simulink model "DPWMA_17_Level_Rectifier_Dual_PI"  (R2021b)
settings: Solver=VariableStepAuto  StartTime=0.0  StopTime=0.5  RelTol=1e-3
libraries: spsSeriesRLCBranchLib x51, spsVoltageMeasurementLib x27, spsDiodeLib x24, spsIGBTDiodeLib x24, simulink x24, spsUniversalBridgeLib x24, slpidlib x3, spsACVoltageSourceLib x3, spsCurrentMeasurementLib x2, spsMeanLib x2, spsRMSLib x2, spsTHDLib x1
(part 2 of 3)

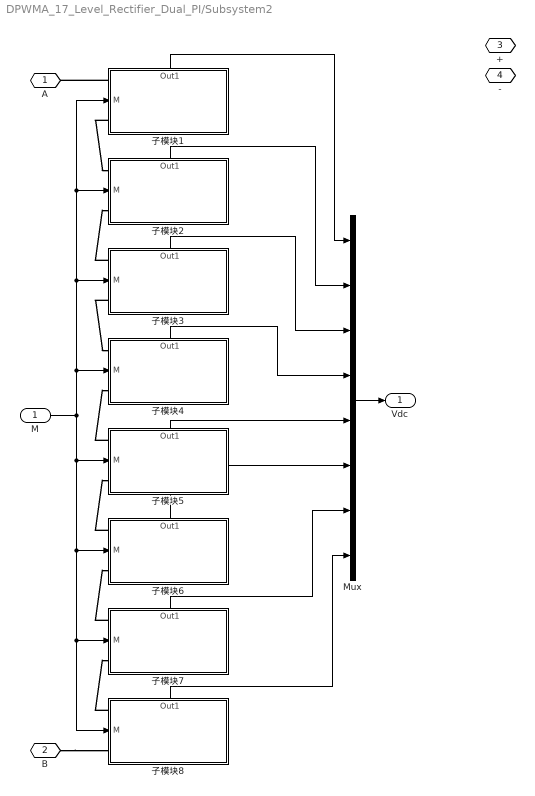
== system DPWMA_17_Level_Rectifier_Dual_PI/Subsystem2 ==
  M : Inport
  Mux : Mux  Inputs=8
  子模块1 : Subsystem
      settings: PortSchema="{\"entries\":[{\"content\":{\"sides\":[{\"content\":{\"connectorIds\":[\"LConn1\",\"LConn2\"]},\"type\":\"ConnectorPlacement.EquallySpacedRectSide\",\"uuid\":\"47187a24-6853-42ac-9ad9-0df0e1360fae\"},{\"content\":{\"connectorIds\":[\"RConn1\",\"In1\",\"RConn2\"],\"side\":\"RIGHT\"},\"type\":\"ConnectorPlacement.EquallySpacedRectSide\",\"uuid\":\"b3504369-b235-4116-9b9b-167bd6b76527\"},{\"content\":{\"connectorIds\":[\"Out1\"],\"side\":\"TOP\"},\"type\":\"ConnectorPlacement.EquallySpacedRectSide\",\"uuid\":\"5cb205b4-da18-4f20-b3d4-22846a9c2236\"},{\"content\":{\"connectorIds\":[],\"side\":\"BOTTOM\"},\"type\":\"ConnectorPlacement.EquallySpacedRectSide\",\"uuid\":\"4e548a82-6bdf-470e-8572-00c7c8855d01\"}]},\"type\":\"ConnectorPlacement.EquallySpacedConnector\",\"uuid\":\"b00ba750-ea4b-4b64-a122-5cbc9e899126\"}],\"packageUris\":[\"http://schema.mathworks.com/mf0/Connector/R2020b\"],\"version\":\"1.0\"}"
  子模块2 : Subsystem
      settings: PortSchema="{\"entries\":[{\"content\":{\"sides\":[{\"content\":{\"connectorIds\":[\"LConn1\",\"LConn2\"]},\"type\":\"ConnectorPlacement.EquallySpacedRectSide\",\"uuid\":\"47187a24-6853-42ac-9ad9-0df0e1360fae\"},{\"content\":{\"connectorIds\":[\"RConn1\",\"In1\",\"RConn2\"],\"side\":\"RIGHT\"},\"type\":\"ConnectorPlacement.EquallySpacedRectSide\",\"uuid\":\"b3504369-b235-4116-9b9b-167bd6b76527\"},{\"content\":{\"connectorIds\":[\"Out1\"],\"side\":\"TOP\"},\"type\":\"ConnectorPlacement.EquallySpacedRectSide\",\"uuid\":\"5cb205b4-da18-4f20-b3d4-22846a9c2236\"},{\"content\":{\"connectorIds\":[],\"side\":\"BOTTOM\"},\"type\":\"ConnectorPlacement.EquallySpacedRectSide\",\"uuid\":\"4e548a82-6bdf-470e-8572-00c7c8855d01\"}]},\"type\":\"ConnectorPlacement.EquallySpacedConnector\",\"uuid\":\"b00ba750-ea4b-4b64-a122-5cbc9e899126\"}],\"packageUris\":[\"http://schema.mathworks.com/mf0/Connector/R2020b\"],\"version\":\"1.0\"}"
  子模块3 : Subsystem
      settings: PortSchema="{\"entries\":[{\"content\":{\"sides\":[{\"content\":{\"connectorIds\":[\"LConn1\",\"LConn2\"]},\"type\":\"ConnectorPlacement.EquallySpacedRectSide\",\"uuid\":\"47187a24-6853-42ac-9ad9-0df0e1360fae\"},{\"content\":{\"connectorIds\":[\"RConn1\",\"In1\",\"RConn2\"],\"side\":\"RIGHT\"},\"type\":\"ConnectorPlacement.EquallySpacedRectSide\",\"uuid\":\"b3504369-b235-4116-9b9b-167bd6b76527\"},{\"content\":{\"connectorIds\":[\"Out1\"],\"side\":\"TOP\"},\"type\":\"ConnectorPlacement.EquallySpacedRectSide\",\"uuid\":\"5cb205b4-da18-4f20-b3d4-22846a9c2236\"},{\"content\":{\"connectorIds\":[],\"side\":\"BOTTOM\"},\"type\":\"ConnectorPlacement.EquallySpacedRectSide\",\"uuid\":\"4e548a82-6bdf-470e-8572-00c7c8855d01\"}]},\"type\":\"ConnectorPlacement.EquallySpacedConnector\",\"uuid\":\"b00ba750-ea4b-4b64-a122-5cbc9e899126\"}],\"packageUris\":[\"http://schema.mathworks.com/mf0/Connector/R2020b\"],\"version\":\"1.0\"}"
  子模块4 : Subsystem
      settings: PortSchema="{\"entries\":[{\"content\":{\"sides\":[{\"content\":{\"connectorIds\":[\"LConn1\",\"LConn2\"]},\"type\":\"ConnectorPlacement.EquallySpacedRectSide\",\"uuid\":\"47187a24-6853-42ac-9ad9-0df0e1360fae\"},{\"content\":{\"connectorIds\":[\"RConn1\",\"In1\",\"RConn2\"],\"side\":\"RIGHT\"},\"type\":\"ConnectorPlacement.EquallySpacedRectSide\",\"uuid\":\"b3504369-b235-4116-9b9b-167bd6b76527\"},{\"content\":{\"connectorIds\":[\"Out1\"],\"side\":\"TOP\"},\"type\":\"ConnectorPlacement.EquallySpacedRectSide\",\"uuid\":\"5cb205b4-da18-4f20-b3d4-22846a9c2236\"},{\"content\":{\"connectorIds\":[],\"side\":\"BOTTOM\"},\"type\":\"ConnectorPlacement.EquallySpacedRectSide\",\"uuid\":\"4e548a82-6bdf-470e-8572-00c7c8855d01\"}]},\"type\":\"ConnectorPlacement.EquallySpacedConnector\",\"uuid\":\"b00ba750-ea4b-4b64-a122-5cbc9e899126\"}],\"packageUris\":[\"http://schema.mathworks.com/mf0/Connector/R2020b\"],\"version\":\"1.0\"}"
  子模块5 : Subsystem
      settings: PortSchema="{\"entries\":[{\"content\":{\"sides\":[{\"content\":{\"connectorIds\":[\"LConn1\",\"LConn2\"]},\"type\":\"ConnectorPlacement.EquallySpacedRectSide\",\"uuid\":\"47187a24-6853-42ac-9ad9-0df0e1360fae\"},{\"content\":{\"connectorIds\":[\"RConn1\",\"In1\",\"RConn2\"],\"side\":\"RIGHT\"},\"type\":\"ConnectorPlacement.EquallySpacedRectSide\",\"uuid\":\"b3504369-b235-4116-9b9b-167bd6b76527\"},{\"content\":{\"connectorIds\":[\"Out1\"],\"side\":\"TOP\"},\"type\":\"ConnectorPlacement.EquallySpacedRectSide\",\"uuid\":\"5cb205b4-da18-4f20-b3d4-22846a9c2236\"},{\"content\":{\"connectorIds\":[],\"side\":\"BOTTOM\"},\"type\":\"ConnectorPlacement.EquallySpacedRectSide\",\"uuid\":\"4e548a82-6bdf-470e-8572-00c7c8855d01\"}]},\"type\":\"ConnectorPlacement.EquallySpacedConnector\",\"uuid\":\"b00ba750-ea4b-4b64-a122-5cbc9e899126\"}],\"packageUris\":[\"http://schema.mathworks.com/mf0/Connector/R2020b\"],\"version\":\"1.0\"}"
  子模块6 : Subsystem
      settings: PortSchema="{\"entries\":[{\"content\":{\"sides\":[{\"content\":{\"connectorIds\":[\"LConn1\",\"LConn2\"]},\"type\":\"ConnectorPlacement.EquallySpacedRectSide\",\"uuid\":\"47187a24-6853-42ac-9ad9-0df0e1360fae\"},{\"content\":{\"connectorIds\":[\"RConn1\",\"In1\",\"RConn2\"],\"side\":\"RIGHT\"},\"type\":\"ConnectorPlacement.EquallySpacedRectSide\",\"uuid\":\"b3504369-b235-4116-9b9b-167bd6b76527\"},{\"content\":{\"connectorIds\":[\"Out1\"],\"side\":\"TOP\"},\"type\":\"ConnectorPlacement.EquallySpacedRectSide\",\"uuid\":\"5cb205b4-da18-4f20-b3d4-22846a9c2236\"},{\"content\":{\"connectorIds\":[],\"side\":\"BOTTOM\"},\"type\":\"ConnectorPlacement.EquallySpacedRectSide\",\"uuid\":\"4e548a82-6bdf-470e-8572-00c7c8855d01\"}]},\"type\":\"ConnectorPlacement.EquallySpacedConnector\",\"uuid\":\"b00ba750-ea4b-4b64-a122-5cbc9e899126\"}],\"packageUris\":[\"http://schema.mathworks.com/mf0/Connector/R2020b\"],\"version\":\"1.0\"}"
  子模块7 : Subsystem
      settings: PortSchema="{\"entries\":[{\"content\":{\"sides\":[{\"content\":{\"connectorIds\":[\"LConn1\",\"LConn2\"]},\"type\":\"ConnectorPlacement.EquallySpacedRectSide\",\"uuid\":\"47187a24-6853-42ac-9ad9-0df0e1360fae\"},{\"content\":{\"connectorIds\":[\"RConn1\",\"In1\",\"RConn2\"],\"side\":\"RIGHT\"},\"type\":\"ConnectorPlacement.EquallySpacedRectSide\",\"uuid\":\"b3504369-b235-4116-9b9b-167bd6b76527\"},{\"content\":{\"connectorIds\":[\"Out1\"],\"side\":\"TOP\"},\"type\":\"ConnectorPlacement.EquallySpacedRectSide\",\"uuid\":\"5cb205b4-da18-4f20-b3d4-22846a9c2236\"},{\"content\":{\"connectorIds\":[],\"side\":\"BOTTOM\"},\"type\":\"ConnectorPlacement.EquallySpacedRectSide\",\"uuid\":\"4e548a82-6bdf-470e-8572-00c7c8855d01\"}]},\"type\":\"ConnectorPlacement.EquallySpacedConnector\",\"uuid\":\"b00ba750-ea4b-4b64-a122-5cbc9e899126\"}],\"packageUris\":[\"http://schema.mathworks.com/mf0/Connector/R2020b\"],\"version\":\"1.0\"}"
  子模块8 : Subsystem
      settings: PortSchema="{\"entries\":[{\"content\":{\"sides\":[{\"content\":{\"connectorIds\":[\"LConn1\",\"LConn2\"]},\"type\":\"ConnectorPlacement.EquallySpacedRectSide\",\"uuid\":\"47187a24-6853-42ac-9ad9-0df0e1360fae\"},{\"content\":{\"connectorIds\":[\"RConn1\",\"In1\",\"RConn2\"],\"side\":\"RIGHT\"},\"type\":\"ConnectorPlacement.EquallySpacedRectSide\",\"uuid\":\"b3504369-b235-4116-9b9b-167bd6b76527\"},{\"content\":{\"connectorIds\":[\"Out1\"],\"side\":\"TOP\"},\"type\":\"ConnectorPlacement.EquallySpacedRectSide\",\"uuid\":\"5cb205b4-da18-4f20-b3d4-22846a9c2236\"},{\"content\":{\"connectorIds\":[],\"side\":\"BOTTOM\"},\"type\":\"ConnectorPlacement.EquallySpacedRectSide\",\"uuid\":\"4e548a82-6bdf-470e-8572-00c7c8855d01\"}]},\"type\":\"ConnectorPlacement.EquallySpacedConnector\",\"uuid\":\"b00ba750-ea4b-4b64-a122-5cbc9e899126\"}],\"packageUris\":[\"http://schema.mathworks.com/mf0/Connector/R2020b\"],\"version\":\"1.0\"}"
  A : PMIOPort  Side=Left
  B : PMIOPort  Port=2  Side=Left
  + : PMIOPort  Port=3  Side=Right
  - : PMIOPort  Port=4  Side=Right
  Vdc : Outport
  wires:
  子模块3/1(Out1) -> Mux/3
  子模块1/1(Out1) -> Mux/1
  子模块2/1(Out1) -> Mux/2
  子模块4/1(Out1) -> Mux/4
  Mux/1 -> Vdc/1
  M/1 -> 子模块8/1(M), 子模块7/1(M), 子模块6/1(M), 子模块5/1(M), 子模块1/1(M), 子模块2/1(M), 子模块3/1(M), 子模块4/1(M)
  子模块8/1(Out1) -> Mux/8
  子模块6/1(Out1) -> Mux/6
  子模块7/1(Out1) -> Mux/7
  子模块5/1(Out1) -> Mux/5
  connections:
  子模块1/RConn2 -- 子模块2/RConn1
  子模块1/RConn1 -- A/RConn1
  子模块3/RConn1 -- 子模块2/RConn2
  子模块3/RConn2 -- 子模块4/RConn1
  B/RConn1 -- 子模块8/RConn2
  子模块8/RConn1 -- 子模块7/RConn2
  子模块7/RConn1 -- 子模块6/RConn2
  子模块6/RConn1 -- 子模块5/RConn2
  子模块5/RConn1 -- 子模块4/RConn2

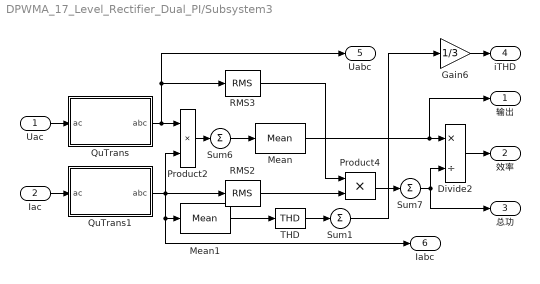
== system DPWMA_17_Level_Rectifier_Dual_PI/Subsystem3 ==
  Uac : Inport
  Iac : Inport  Port=2
  Divide2 : Product  Inputs=*/
  Gain6 : Gain  Gain=1/3
  Mean : spsMeanLib/Mean  Freq=100  Vinit=0  Ts=0
  Mean1 : spsMeanLib/Mean  Freq=20000  Vinit=0  Ts=0
  Product2 : Product
  Product4 : Product
  QuTrans : Subsystem
      settings: PortSchema="{\"entries\":[{\"content\":{\"sides\":[{\"content\":{\"connectorIds\":[]},\"type\":\"ConnectorPlacement.EquallySpacedRectSide\",\"uuid\":\"58c40194-9a95-4e39-952e-f878bde7484e\"},{\"content\":{\"connectorIds\":[],\"side\":\"RIGHT\"},\"type\":\"ConnectorPlacement.EquallySpacedRectSide\",\"uuid\":\"f51692e8-3ff2-4d72-808d-3667196a4526\"},{\"content\":{\"connectorIds\":[\"In1\"],\"side\":\"TOP\"},\"type\":\"ConnectorPlacement.EquallySpacedRectSide\",\"uuid\":\"0aab136b-5da5-45c4-8998-999ebe8b7f2f\"},{\"content\":{\"connectorIds\":[\"Out1\"],\"side\":\"BOTTOM\"},\"type\":\"ConnectorPlacement.EquallySpacedRectSide\",\"uuid\":\"185ce796-68e2-4136-8080-97dc86d2ba54\"}]},\"type\":\"ConnectorPlacement.EquallySpacedConnector\",\"uuid\":\"3ef81af7-d426-47fb-88e3-e33e58eebb83\"}],\"packageUris\":[\"http://schema.mathworks.com/mf0/Connector/R2020b\"],\"version\":\"1.0\"}"
  QuTrans1 : Subsystem
      settings: PortSchema="{\"entries\":[{\"content\":{\"sides\":[{\"content\":{\"connectorIds\":[]},\"type\":\"ConnectorPlacement.EquallySpacedRectSide\",\"uuid\":\"58c40194-9a95-4e39-952e-f878bde7484e\"},{\"content\":{\"connectorIds\":[],\"side\":\"RIGHT\"},\"type\":\"ConnectorPlacement.EquallySpacedRectSide\",\"uuid\":\"f51692e8-3ff2-4d72-808d-3667196a4526\"},{\"content\":{\"connectorIds\":[\"In1\"],\"side\":\"TOP\"},\"type\":\"ConnectorPlacement.EquallySpacedRectSide\",\"uuid\":\"0aab136b-5da5-45c4-8998-999ebe8b7f2f\"},{\"content\":{\"connectorIds\":[\"Out1\"],\"side\":\"BOTTOM\"},\"type\":\"ConnectorPlacement.EquallySpacedRectSide\",\"uuid\":\"185ce796-68e2-4136-8080-97dc86d2ba54\"}]},\"type\":\"ConnectorPlacement.EquallySpacedConnector\",\"uuid\":\"3ef81af7-d426-47fb-88e3-e33e58eebb83\"}],\"packageUris\":[\"http://schema.mathworks.com/mf0/Connector/R2020b\"],\"version\":\"1.0\"}"
  RMS2 : spsRMSLib/RMS  TrueRMS=on  Freq=50  RMSInit=0  Ts=0
  RMS3 : spsRMSLib/RMS  TrueRMS=on  Freq=50  RMSInit=0  Ts=0
  Sum1 : Sum  Inputs=+
  Sum6 : Sum  Inputs=+
  Sum7 : Sum  Inputs=+
  THD : spsTHDLib/THD  Freq=50  Ts=0
      settings: SourceProductBaseCode=PS
  输出 : Outport
  效率 : Outport  Port=2
  总功 : Outport  Port=3
  iTHD : Outport  Port=4
  Uabc : Outport  Port=5
  Iabc : Outport  Port=6
  wires:
  RMS3/1 -> Product4/1
  Product4/1 -> Sum7/1
  Sum6/1 -> Mean/1
  Product2/1 -> Sum6/1
  Divide2/1 -> 效率/1
  RMS2/1 -> Product4/2
  Sum1/1 -> Gain6/1
  Gain6/1 -> iTHD/1
  Sum7/1 -> 总功/1, Divide2/2
  Mean/1 -> 输出/1, Divide2/1
  THD/1 -> Sum1/1
  Mean1/1 -> THD/1
  Uac/1 -> QuTrans/1(ac)
  Iac/1 -> QuTrans1/1(ac)
  QuTrans1/1(abc) -> Product2/2, Iabc/1, Mean1/1, RMS2/1
  QuTrans/1(abc) -> Uabc/1, RMS3/1, Product2/1

== system DPWMA_17_Level_Rectifier_Dual_PI/三相电源 ==
  5.7KV2 : spsACVoltageSourceLib/AC Voltage Source  Amplitude=5770*1.414  Phase=120  Frequency=50  SampleTime=0  Measurements=None  BusType=swing  Pref=10e3  Qref=0  Qmin=-inf  Qmax=+inf
  5.7kV : spsACVoltageSourceLib/AC Voltage Source  Amplitude=5770*1.414  Phase=0  Frequency=50  SampleTime=0  Measurements=None  BusType=swing  Pref=10e3  Qref=0  Qmin=-inf  Qmax=+inf
  5.7kV1 : spsACVoltageSourceLib/AC Voltage Source  Amplitude=5770*1.414  Phase=240  Frequency=50  SampleTime=0  Measurements=None  BusType=swing  Pref=10e3  Qref=0  Qmin=-inf  Qmax=+inf
  A : PMIOPort  Side=Right
  B : PMIOPort  Port=2  Side=Right
  C : PMIOPort  Port=3  Side=Right
  N : PMIOPort  Port=4  Side=Right
  connections:
  5.7kV/LConn1 -- N/RConn1 -- 5.7KV2/LConn1 -- 5.7kV1/LConn1
  A/RConn1 -- 5.7kV/RConn1
  B/RConn1 -- 5.7kV1/RConn1
  C/RConn1 -- 5.7KV2/RConn1

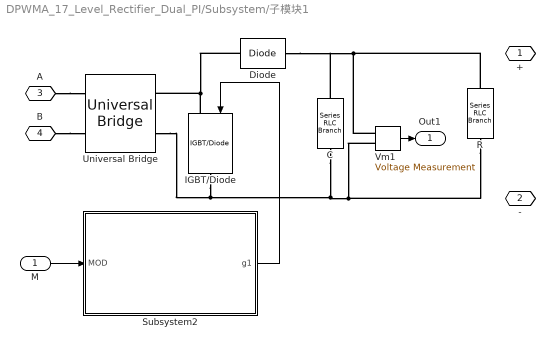
== system DPWMA_17_Level_Rectifier_Dual_PI/Subsystem/子模块1 ==
  M : Inport
  C : spsSeriesRLCBranchLib/Series RLC Branch  LConnTagsString=__new0  RConnTagsString=__new0  BranchType=C  Resistance=0  Inductance=0  SetiL0=off  InitialCurrent=0  Capacitance=4e-3  Setx0=on  InitialVoltage=1000  Measurements=None
  Diode : spsDiodeLib/Diode  Ron=0.001  Lon=0  Vf=2  IC=0  UseSnubber=0  Rs=1e6  Cs=2e-9  Measurements=off
  IGBT/Diode : spsIGBTDiodeLib/IGBT//Diode  Ron=1e-3  Rs=1e5  Cs=inf  Measurements=off
  R : spsSeriesRLCBranchLib/Series RLC Branch  LConnTagsString=__new0  RConnTagsString=__new0  BranchType=R  Resistance=15  Inductance=0  SetiL0=off  InitialCurrent=0  Capacitance=2e-3  Setx0=on  InitialVoltage=311  Measurements=None
  Subsystem2 : Subsystem
  Universal Bridge : spsUniversalBridgeLib/Universal Bridge  Arms=2  SnubberResistance=0.01  SnubberCapacitance=1e-8  Device=Diodes  Ron=1e-3  Lon=0  ForwardVoltages="[  0  0  ]"  ForwardVoltage=3  GTOparameters=[ 10e-6 , 20e-6 ]  IGBTparameters=[ 1e-6 , 2e-6 ]  Measurements=None  Measurements_2=None  converterType=Rectifier
  Vm1 : spsVoltageMeasurementLib/Voltage Measurement  PhasorSimulation=off  OutputType=Complex  PSBequivalent=0
  + : PMIOPort  Side=Left
  - : PMIOPort  Port=2  Side=Left
  A : PMIOPort  Port=3  Side=Right
  B : PMIOPort  Port=4  Side=Right
  Out1 : Outport
  wires:
  Vm1/1 -> Out1/1
  M/1 -> Subsystem2/1(MOD)
  Subsystem2/1(g1) -> IGBT/Diode/1
  connections:
  Universal Bridge/RConn2 -- Vm1/LConn2 -- R/RConn1 -- C/RConn1 -- IGBT/Diode/RConn1
  Vm1/LConn1 -- R/LConn1 -- C/LConn1 -- Diode/RConn1
  A/RConn1 -- Universal Bridge/LConn1
  B/RConn1 -- Universal Bridge/LConn2
  IGBT/Diode/LConn1 -- Universal Bridge/RConn1 -- Diode/LConn1

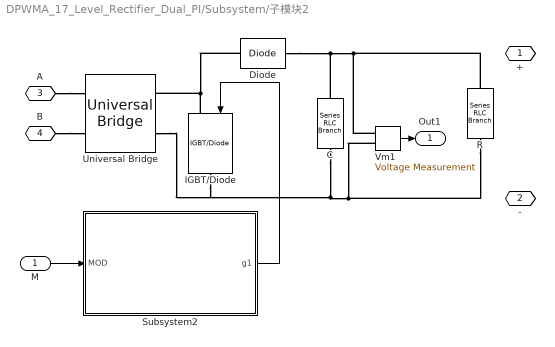
== system DPWMA_17_Level_Rectifier_Dual_PI/Subsystem/子模块2 ==
  M : Inport
  C : spsSeriesRLCBranchLib/Series RLC Branch  LConnTagsString=__new0  RConnTagsString=__new0  BranchType=C  Resistance=0  Inductance=0  SetiL0=off  InitialCurrent=0  Capacitance=4e-3  Setx0=on  InitialVoltage=1000  Measurements=None
  Diode : spsDiodeLib/Diode  Ron=0.001  Lon=0  Vf=2  IC=0  UseSnubber=0  Rs=1e6  Cs=2e-9  Measurements=off
  IGBT/Diode : spsIGBTDiodeLib/IGBT//Diode  Ron=1e-3  Rs=1e5  Cs=inf  Measurements=off
  R : spsSeriesRLCBranchLib/Series RLC Branch  LConnTagsString=__new0  RConnTagsString=__new0  BranchType=R  Resistance=15  Inductance=0  SetiL0=off  InitialCurrent=0  Capacitance=2e-3  Setx0=on  InitialVoltage=311  Measurements=None
  Subsystem2 : Subsystem
  Universal Bridge : spsUniversalBridgeLib/Universal Bridge  Arms=2  SnubberResistance=0.01  SnubberCapacitance=1e-8  Device=Diodes  Ron=1e-3  Lon=0  ForwardVoltages="[  0  0  ]"  ForwardVoltage=3  GTOparameters=[ 10e-6 , 20e-6 ]  IGBTparameters=[ 1e-6 , 2e-6 ]  Measurements=None  Measurements_2=None  converterType=Rectifier
  Vm1 : spsVoltageMeasurementLib/Voltage Measurement  PhasorSimulation=off  OutputType=Complex  PSBequivalent=0
  + : PMIOPort  Side=Left
  - : PMIOPort  Port=2  Side=Left
  A : PMIOPort  Port=3  Side=Right
  B : PMIOPort  Port=4  Side=Right
  Out1 : Outport
  wires:
  Vm1/1 -> Out1/1
  M/1 -> Subsystem2/1(MOD)
  Subsystem2/1(g1) -> IGBT/Diode/1
  connections:
  Vm1/LConn2 -- IGBT/Diode/RConn1 -- Universal Bridge/RConn2 -- C/RConn1 -- R/RConn1
  C/LConn1 -- Diode/RConn1 -- Vm1/LConn1 -- R/LConn1
  A/RConn1 -- Universal Bridge/LConn1
  B/RConn1 -- Universal Bridge/LConn2
  IGBT/Diode/LConn1 -- Diode/LConn1 -- Universal Bridge/RConn1

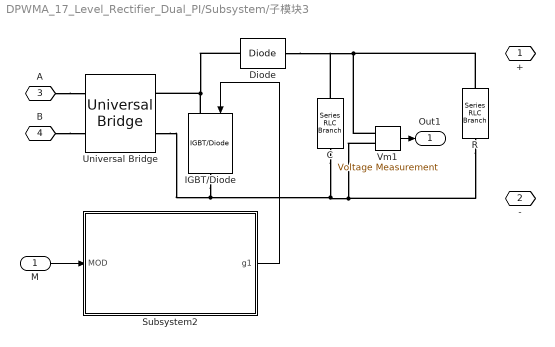
== system DPWMA_17_Level_Rectifier_Dual_PI/Subsystem/子模块3 ==
  M : Inport
  C : spsSeriesRLCBranchLib/Series RLC Branch  LConnTagsString=__new0  RConnTagsString=__new0  BranchType=C  Resistance=0  Inductance=0  SetiL0=off  InitialCurrent=0  Capacitance=4e-3  Setx0=on  InitialVoltage=1000  Measurements=None
  Diode : spsDiodeLib/Diode  Ron=0.001  Lon=0  Vf=2  IC=0  UseSnubber=0  Rs=1e6  Cs=2e-9  Measurements=off
  IGBT/Diode : spsIGBTDiodeLib/IGBT//Diode  Ron=1e-3  Rs=1e5  Cs=inf  Measurements=off
  R : spsSeriesRLCBranchLib/Series RLC Branch  LConnTagsString=__new0  RConnTagsString=__new0  BranchType=R  Resistance=15  Inductance=0  SetiL0=off  InitialCurrent=0  Capacitance=2e-3  Setx0=on  InitialVoltage=311  Measurements=None
  Subsystem2 : Subsystem
  Universal Bridge : spsUniversalBridgeLib/Universal Bridge  Arms=2  SnubberResistance=0.01  SnubberCapacitance=1e-8  Device=Diodes  Ron=1e-3  Lon=0  ForwardVoltages="[  0  0  ]"  ForwardVoltage=3  GTOparameters=[ 10e-6 , 20e-6 ]  IGBTparameters=[ 1e-6 , 2e-6 ]  Measurements=None  Measurements_2=None  converterType=Rectifier
  Vm1 : spsVoltageMeasurementLib/Voltage Measurement  PhasorSimulation=off  OutputType=Complex  PSBequivalent=0
  + : PMIOPort  Side=Left
  - : PMIOPort  Port=2  Side=Left
  A : PMIOPort  Port=3  Side=Right
  B : PMIOPort  Port=4  Side=Right
  Out1 : Outport
  wires:
  Subsystem2/1(g1) -> IGBT/Diode/1
  M/1 -> Subsystem2/1(MOD)
  Vm1/1 -> Out1/1
  connections:
  Diode/LConn1 -- Universal Bridge/RConn1 -- IGBT/Diode/LConn1
  B/RConn1 -- Universal Bridge/LConn2
  A/RConn1 -- Universal Bridge/LConn1
  Diode/RConn1 -- C/LConn1 -- R/LConn1 -- Vm1/LConn1
  IGBT/Diode/RConn1 -- C/RConn1 -- R/RConn1 -- Vm1/LConn2 -- Universal Bridge/RConn2

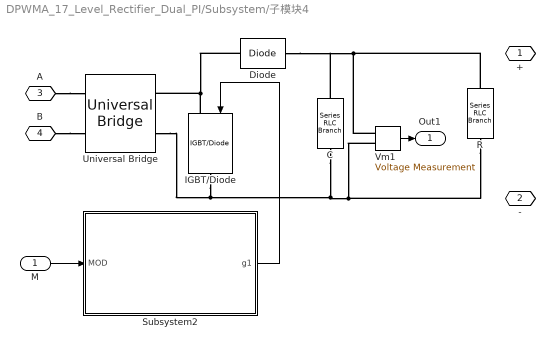
== system DPWMA_17_Level_Rectifier_Dual_PI/Subsystem/子模块4 ==
  M : Inport
  C : spsSeriesRLCBranchLib/Series RLC Branch  LConnTagsString=__new0  RConnTagsString=__new0  BranchType=C  Resistance=0  Inductance=0  SetiL0=off  InitialCurrent=0  Capacitance=4e-3  Setx0=on  InitialVoltage=1000  Measurements=None
  Diode : spsDiodeLib/Diode  Ron=0.001  Lon=0  Vf=2  IC=0  UseSnubber=0  Rs=1e6  Cs=2e-9  Measurements=off
  IGBT/Diode : spsIGBTDiodeLib/IGBT//Diode  Ron=1e-3  Rs=1e5  Cs=inf  Measurements=off
  R : spsSeriesRLCBranchLib/Series RLC Branch  LConnTagsString=__new0  RConnTagsString=__new0  BranchType=R  Resistance=15  Inductance=0  SetiL0=off  InitialCurrent=0  Capacitance=2e-3  Setx0=on  InitialVoltage=311  Measurements=None
  Subsystem2 : Subsystem
  Universal Bridge : spsUniversalBridgeLib/Universal Bridge  Arms=2  SnubberResistance=0.01  SnubberCapacitance=1e-8  Device=Diodes  Ron=1e-3  Lon=0  ForwardVoltages="[  0  0  ]"  ForwardVoltage=3  GTOparameters=[ 10e-6 , 20e-6 ]  IGBTparameters=[ 1e-6 , 2e-6 ]  Measurements=None  Measurements_2=None  converterType=Rectifier
  Vm1 : spsVoltageMeasurementLib/Voltage Measurement  PhasorSimulation=off  OutputType=Complex  PSBequivalent=0
  + : PMIOPort  Side=Left
  - : PMIOPort  Port=2  Side=Left
  A : PMIOPort  Port=3  Side=Right
  B : PMIOPort  Port=4  Side=Right
  Out1 : Outport
  wires:
  Vm1/1 -> Out1/1
  M/1 -> Subsystem2/1(MOD)
  Subsystem2/1(g1) -> IGBT/Diode/1
  connections:
  Universal Bridge/RConn2 -- Vm1/LConn2 -- R/RConn1 -- C/RConn1 -- IGBT/Diode/RConn1
  Vm1/LConn1 -- R/LConn1 -- C/LConn1 -- Diode/RConn1
  A/RConn1 -- Universal Bridge/LConn1
  B/RConn1 -- Universal Bridge/LConn2
  IGBT/Diode/LConn1 -- Universal Bridge/RConn1 -- Diode/LConn1

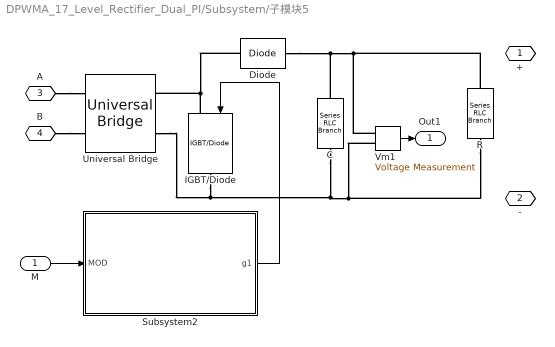
== system DPWMA_17_Level_Rectifier_Dual_PI/Subsystem/子模块5 ==
  M : Inport
  C : spsSeriesRLCBranchLib/Series RLC Branch  LConnTagsString=__new0  RConnTagsString=__new0  BranchType=C  Resistance=0  Inductance=0  SetiL0=off  InitialCurrent=0  Capacitance=4e-3  Setx0=on  InitialVoltage=1000  Measurements=None
  Diode : spsDiodeLib/Diode  Ron=0.001  Lon=0  Vf=2  IC=0  UseSnubber=0  Rs=1e6  Cs=2e-9  Measurements=off
  IGBT/Diode : spsIGBTDiodeLib/IGBT//Diode  Ron=1e-3  Rs=1e5  Cs=inf  Measurements=off
  R : spsSeriesRLCBranchLib/Series RLC Branch  LConnTagsString=__new0  RConnTagsString=__new0  BranchType=R  Resistance=15  Inductance=0  SetiL0=off  InitialCurrent=0  Capacitance=2e-3  Setx0=on  InitialVoltage=311  Measurements=None
  Subsystem2 : Subsystem
  Universal Bridge : spsUniversalBridgeLib/Universal Bridge  Arms=2  SnubberResistance=0.01  SnubberCapacitance=1e-8  Device=Diodes  Ron=1e-3  Lon=0  ForwardVoltages="[  0  0  ]"  ForwardVoltage=3  GTOparameters=[ 10e-6 , 20e-6 ]  IGBTparameters=[ 1e-6 , 2e-6 ]  Measurements=None  Measurements_2=None  converterType=Rectifier
  Vm1 : spsVoltageMeasurementLib/Voltage Measurement  PhasorSimulation=off  OutputType=Complex  PSBequivalent=0
  + : PMIOPort  Side=Left
  - : PMIOPort  Port=2  Side=Left
  A : PMIOPort  Port=3  Side=Right
  B : PMIOPort  Port=4  Side=Right
  Out1 : Outport
  wires:
  Subsystem2/1(g1) -> IGBT/Diode/1
  M/1 -> Subsystem2/1(MOD)
  Vm1/1 -> Out1/1
  connections:
  Diode/LConn1 -- Universal Bridge/RConn1 -- IGBT/Diode/LConn1
  B/RConn1 -- Universal Bridge/LConn2
  A/RConn1 -- Universal Bridge/LConn1
  Diode/RConn1 -- C/LConn1 -- R/LConn1 -- Vm1/LConn1
  IGBT/Diode/RConn1 -- C/RConn1 -- R/RConn1 -- Vm1/LConn2 -- Universal Bridge/RConn2

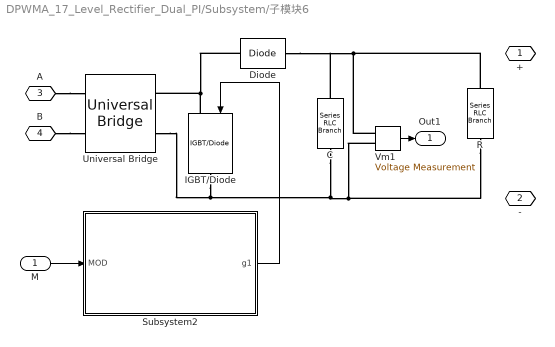
== system DPWMA_17_Level_Rectifier_Dual_PI/Subsystem/子模块6 ==
  M : Inport
  C : spsSeriesRLCBranchLib/Series RLC Branch  LConnTagsString=__new0  RConnTagsString=__new0  BranchType=C  Resistance=0  Inductance=0  SetiL0=off  InitialCurrent=0  Capacitance=4e-3  Setx0=on  InitialVoltage=1000  Measurements=None
  Diode : spsDiodeLib/Diode  Ron=0.001  Lon=0  Vf=2  IC=0  UseSnubber=0  Rs=1e6  Cs=2e-9  Measurements=off
  IGBT/Diode : spsIGBTDiodeLib/IGBT//Diode  Ron=1e-3  Rs=1e5  Cs=inf  Measurements=off
  R : spsSeriesRLCBranchLib/Series RLC Branch  LConnTagsString=__new0  RConnTagsString=__new0  BranchType=R  Resistance=15  Inductance=0  SetiL0=off  InitialCurrent=0  Capacitance=2e-3  Setx0=on  InitialVoltage=311  Measurements=None
  Subsystem2 : Subsystem
  Universal Bridge : spsUniversalBridgeLib/Universal Bridge  Arms=2  SnubberResistance=0.01  SnubberCapacitance=1e-8  Device=Diodes  Ron=1e-3  Lon=0  ForwardVoltages="[  0  0  ]"  ForwardVoltage=3  GTOparameters=[ 10e-6 , 20e-6 ]  IGBTparameters=[ 1e-6 , 2e-6 ]  Measurements=None  Measurements_2=None  converterType=Rectifier
  Vm1 : spsVoltageMeasurementLib/Voltage Measurement  PhasorSimulation=off  OutputType=Complex  PSBequivalent=0
  + : PMIOPort  Side=Left
  - : PMIOPort  Port=2  Side=Left
  A : PMIOPort  Port=3  Side=Right
  B : PMIOPort  Port=4  Side=Right
  Out1 : Outport
  wires:
  Subsystem2/1(g1) -> IGBT/Diode/1
  M/1 -> Subsystem2/1(MOD)
  Vm1/1 -> Out1/1
  connections:
  Diode/LConn1 -- Universal Bridge/RConn1 -- IGBT/Diode/LConn1
  B/RConn1 -- Universal Bridge/LConn2
  A/RConn1 -- Universal Bridge/LConn1
  Diode/RConn1 -- C/LConn1 -- R/LConn1 -- Vm1/LConn1
  IGBT/Diode/RConn1 -- C/RConn1 -- R/RConn1 -- Vm1/LConn2 -- Universal Bridge/RConn2

== system DPWMA_17_Level_Rectifier_Dual_PI/Subsystem/子模块7 ==
  M : Inport
  C : spsSeriesRLCBranchLib/Series RLC Branch  LConnTagsString=__new0  RConnTagsString=__new0  BranchType=C  Resistance=0  Inductance=0  SetiL0=off  InitialCurrent=0  Capacitance=4e-3  Setx0=on  InitialVoltage=1000  Measurements=None
  Diode : spsDiodeLib/Diode  Ron=0.001  Lon=0  Vf=2  IC=0  UseSnubber=0  Rs=1e6  Cs=2e-9  Measurements=off
  IGBT/Diode : spsIGBTDiodeLib/IGBT//Diode  Ron=1e-3  Rs=1e5  Cs=inf  Measurements=off
  R : spsSeriesRLCBranchLib/Series RLC Branch  LConnTagsString=__new0  RConnTagsString=__new0  BranchType=R  Resistance=15  Inductance=0  SetiL0=off  InitialCurrent=0  Capacitance=2e-3  Setx0=on  InitialVoltage=311  Measurements=None
  Subsystem2 : Subsystem
  Universal Bridge : spsUniversalBridgeLib/Universal Bridge  Arms=2  SnubberResistance=0.01  SnubberCapacitance=1e-8  Device=Diodes  Ron=1e-3  Lon=0  ForwardVoltages="[  0  0  ]"  ForwardVoltage=3  GTOparameters=[ 10e-6 , 20e-6 ]  IGBTparameters=[ 1e-6 , 2e-6 ]  Measurements=None  Measurements_2=None  converterType=Rectifier
  Vm1 : spsVoltageMeasurementLib/Voltage Measurement  PhasorSimulation=off  OutputType=Complex  PSBequivalent=0
  + : PMIOPort  Side=Left
  - : PMIOPort  Port=2  Side=Left
  A : PMIOPort  Port=3  Side=Right
  B : PMIOPort  Port=4  Side=Right
  Out1 : Outport
  wires:
  Vm1/1 -> Out1/1
  M/1 -> Subsystem2/1(MOD)
  Subsystem2/1(g1) -> IGBT/Diode/1
  connections:
  Universal Bridge/RConn2 -- Vm1/LConn2 -- R/RConn1 -- C/RConn1 -- IGBT/Diode/RConn1
  Vm1/LConn1 -- R/LConn1 -- C/LConn1 -- Diode/RConn1
  A/RConn1 -- Universal Bridge/LConn1
  B/RConn1 -- Universal Bridge/LConn2
  IGBT/Diode/LConn1 -- Universal Bridge/RConn1 -- Diode/LConn1

== system DPWMA_17_Level_Rectifier_Dual_PI/Subsystem/子模块8 ==
  M : Inport
  C : spsSeriesRLCBranchLib/Series RLC Branch  LConnTagsString=__new0  RConnTagsString=__new0  BranchType=C  Resistance=0  Inductance=0  SetiL0=off  InitialCurrent=0  Capacitance=4e-3  Setx0=on  InitialVoltage=1000  Measurements=None
  Diode : spsDiodeLib/Diode  Ron=0.001  Lon=0  Vf=2  IC=0  UseSnubber=0  Rs=1e6  Cs=2e-9  Measurements=off
  IGBT/Diode : spsIGBTDiodeLib/IGBT//Diode  Ron=1e-3  Rs=1e5  Cs=inf  Measurements=off
  R : spsSeriesRLCBranchLib/Series RLC Branch  LConnTagsString=__new0  RConnTagsString=__new0  BranchType=R  Resistance=15  Inductance=0  SetiL0=off  InitialCurrent=0  Capacitance=2e-3  Setx0=on  InitialVoltage=311  Measurements=None
  Subsystem2 : Subsystem
  Universal Bridge : spsUniversalBridgeLib/Universal Bridge  Arms=2  SnubberResistance=0.01  SnubberCapacitance=1e-8  Device=Diodes  Ron=1e-3  Lon=0  ForwardVoltages="[  0  0  ]"  ForwardVoltage=3  GTOparameters=[ 10e-6 , 20e-6 ]  IGBTparameters=[ 1e-6 , 2e-6 ]  Measurements=None  Measurements_2=None  converterType=Rectifier
  Vm1 : spsVoltageMeasurementLib/Voltage Measurement  PhasorSimulation=off  OutputType=Complex  PSBequivalent=0
  + : PMIOPort  Side=Left
  - : PMIOPort  Port=2  Side=Left
  A : PMIOPort  Port=3  Side=Right
  B : PMIOPort  Port=4  Side=Right
  Out1 : Outport
  wires:
  Subsystem2/1(g1) -> IGBT/Diode/1
  M/1 -> Subsystem2/1(MOD)
  Vm1/1 -> Out1/1
  connections:
  Diode/LConn1 -- Universal Bridge/RConn1 -- IGBT/Diode/LConn1
  B/RConn1 -- Universal Bridge/LConn2
  A/RConn1 -- Universal Bridge/LConn1
  Diode/RConn1 -- C/LConn1 -- R/LConn1 -- Vm1/LConn1
  IGBT/Diode/RConn1 -- C/RConn1 -- R/RConn1 -- Vm1/LConn2 -- Universal Bridge/RConn2

== system DPWMA_17_Level_Rectifier_Dual_PI/Subsystem1/子模块1 ==
  M : Inport
  C : spsSeriesRLCBranchLib/Series RLC Branch  LConnTagsString=__new0  RConnTagsString=__new0  BranchType=C  Resistance=0  Inductance=0  SetiL0=off  InitialCurrent=0  Capacitance=4e-3  Setx0=on  InitialVoltage=1000  Measurements=None
  Diode : spsDiodeLib/Diode  Ron=0.001  Lon=0  Vf=2  IC=0  UseSnubber=0  Rs=1e6  Cs=2e-9  Measurements=off
  IGBT/Diode : spsIGBTDiodeLib/IGBT//Diode  Ron=1e-3  Rs=1e5  Cs=inf  Measurements=off
  R : spsSeriesRLCBranchLib/Series RLC Branch  LConnTagsString=__new0  RConnTagsString=__new0  BranchType=R  Resistance=15  Inductance=0  SetiL0=off  InitialCurrent=0  Capacitance=2e-3  Setx0=on  InitialVoltage=311  Measurements=None
  Subsystem2 : Subsystem
  Universal Bridge : spsUniversalBridgeLib/Universal Bridge  Arms=2  SnubberResistance=0.01  SnubberCapacitance=1e-8  Device=Diodes  Ron=1e-3  Lon=0  ForwardVoltages="[  0  0  ]"  ForwardVoltage=3  GTOparameters=[ 10e-6 , 20e-6 ]  IGBTparameters=[ 1e-6 , 2e-6 ]  Measurements=None  Measurements_2=None  converterType=Rectifier
  Vm1 : spsVoltageMeasurementLib/Voltage Measurement  PhasorSimulation=off  OutputType=Complex  PSBequivalent=0
  + : PMIOPort  Side=Left
  - : PMIOPort  Port=2  Side=Left
  A : PMIOPort  Port=3  Side=Right
  B : PMIOPort  Port=4  Side=Right
  Out1 : Outport
  wires:
  Subsystem2/1(g1) -> IGBT/Diode/1
  M/1 -> Subsystem2/1(MOD)
  Vm1/1 -> Out1/1
  connections:
  Diode/LConn1 -- Universal Bridge/RConn1 -- IGBT/Diode/LConn1
  B/RConn1 -- Universal Bridge/LConn2
  A/RConn1 -- Universal Bridge/LConn1
  Diode/RConn1 -- C/LConn1 -- R/LConn1 -- Vm1/LConn1
  IGBT/Diode/RConn1 -- C/RConn1 -- R/RConn1 -- Vm1/LConn2 -- Universal Bridge/RConn2

== system DPWMA_17_Level_Rectifier_Dual_PI/Subsystem1/子模块2 ==
  M : Inport
  C : spsSeriesRLCBranchLib/Series RLC Branch  LConnTagsString=__new0  RConnTagsString=__new0  BranchType=C  Resistance=0  Inductance=0  SetiL0=off  InitialCurrent=0  Capacitance=4e-3  Setx0=on  InitialVoltage=1000  Measurements=None
  Diode : spsDiodeLib/Diode  Ron=0.001  Lon=0  Vf=2  IC=0  UseSnubber=0  Rs=1e6  Cs=2e-9  Measurements=off
  IGBT/Diode : spsIGBTDiodeLib/IGBT//Diode  Ron=1e-3  Rs=1e5  Cs=inf  Measurements=off
  R : spsSeriesRLCBranchLib/Series RLC Branch  LConnTagsString=__new0  RConnTagsString=__new0  BranchType=R  Resistance=15  Inductance=0  SetiL0=off  InitialCurrent=0  Capacitance=2e-3  Setx0=on  InitialVoltage=311  Measurements=None
  Subsystem2 : Subsystem
  Universal Bridge : spsUniversalBridgeLib/Universal Bridge  Arms=2  SnubberResistance=0.01  SnubberCapacitance=1e-8  Device=Diodes  Ron=1e-3  Lon=0  ForwardVoltages="[  0  0  ]"  ForwardVoltage=3  GTOparameters=[ 10e-6 , 20e-6 ]  IGBTparameters=[ 1e-6 , 2e-6 ]  Measurements=None  Measurements_2=None  converterType=Rectifier
  Vm1 : spsVoltageMeasurementLib/Voltage Measurement  PhasorSimulation=off  OutputType=Complex  PSBequivalent=0
  + : PMIOPort  Side=Left
  - : PMIOPort  Port=2  Side=Left
  A : PMIOPort  Port=3  Side=Right
  B : PMIOPort  Port=4  Side=Right
  Out1 : Outport
  wires:
  Subsystem2/1(g1) -> IGBT/Diode/1
  M/1 -> Subsystem2/1(MOD)
  Vm1/1 -> Out1/1
  connections:
  Diode/LConn1 -- Universal Bridge/RConn1 -- IGBT/Diode/LConn1
  B/RConn1 -- Universal Bridge/LConn2
  A/RConn1 -- Universal Bridge/LConn1
  Diode/RConn1 -- C/LConn1 -- R/LConn1 -- Vm1/LConn1
  IGBT/Diode/RConn1 -- C/RConn1 -- R/RConn1 -- Vm1/LConn2 -- Universal Bridge/RConn2

== system DPWMA_17_Level_Rectifier_Dual_PI/Subsystem1/子模块3 ==
  M : Inport
  C : spsSeriesRLCBranchLib/Series RLC Branch  LConnTagsString=__new0  RConnTagsString=__new0  BranchType=C  Resistance=0  Inductance=0  SetiL0=off  InitialCurrent=0  Capacitance=4e-3  Setx0=on  InitialVoltage=1000  Measurements=None
  Diode : spsDiodeLib/Diode  Ron=0.001  Lon=0  Vf=2  IC=0  UseSnubber=0  Rs=1e6  Cs=2e-9  Measurements=off
  IGBT/Diode : spsIGBTDiodeLib/IGBT//Diode  Ron=1e-3  Rs=1e5  Cs=inf  Measurements=off
  R : spsSeriesRLCBranchLib/Series RLC Branch  LConnTagsString=__new0  RConnTagsString=__new0  BranchType=R  Resistance=15  Inductance=0  SetiL0=off  InitialCurrent=0  Capacitance=2e-3  Setx0=on  InitialVoltage=311  Measurements=None
  Subsystem2 : Subsystem
  Universal Bridge : spsUniversalBridgeLib/Universal Bridge  Arms=2  SnubberResistance=0.01  SnubberCapacitance=1e-8  Device=Diodes  Ron=1e-3  Lon=0  ForwardVoltages="[  0  0  ]"  ForwardVoltage=3  GTOparameters=[ 10e-6 , 20e-6 ]  IGBTparameters=[ 1e-6 , 2e-6 ]  Measurements=None  Measurements_2=None  converterType=Rectifier
  Vm1 : spsVoltageMeasurementLib/Voltage Measurement  PhasorSimulation=off  OutputType=Complex  PSBequivalent=0
  + : PMIOPort  Side=Left
  - : PMIOPort  Port=2  Side=Left
  A : PMIOPort  Port=3  Side=Right
  B : PMIOPort  Port=4  Side=Right
  Out1 : Outport
  wires:
  Vm1/1 -> Out1/1
  M/1 -> Subsystem2/1(MOD)
  Subsystem2/1(g1) -> IGBT/Diode/1
  connections:
  Universal Bridge/RConn2 -- Vm1/LConn2 -- R/RConn1 -- C/RConn1 -- IGBT/Diode/RConn1
  Vm1/LConn1 -- R/LConn1 -- C/LConn1 -- Diode/RConn1
  A/RConn1 -- Universal Bridge/LConn1
  B/RConn1 -- Universal Bridge/LConn2
  IGBT/Diode/LConn1 -- Universal Bridge/RConn1 -- Diode/LConn1

== system DPWMA_17_Level_Rectifier_Dual_PI/Subsystem1/子模块4 ==
  M : Inport
  C : spsSeriesRLCBranchLib/Series RLC Branch  LConnTagsString=__new0  RConnTagsString=__new0  BranchType=C  Resistance=0  Inductance=0  SetiL0=off  InitialCurrent=0  Capacitance=4e-3  Setx0=on  InitialVoltage=1000  Measurements=None
  Diode : spsDiodeLib/Diode  Ron=0.001  Lon=0  Vf=2  IC=0  UseSnubber=0  Rs=1e6  Cs=2e-9  Measurements=off
  IGBT/Diode : spsIGBTDiodeLib/IGBT//Diode  Ron=1e-3  Rs=1e5  Cs=inf  Measurements=off
  R : spsSeriesRLCBranchLib/Series RLC Branch  LConnTagsString=__new0  RConnTagsString=__new0  BranchType=R  Resistance=15  Inductance=0  SetiL0=off  InitialCurrent=0  Capacitance=2e-3  Setx0=on  InitialVoltage=311  Measurements=None
  Subsystem2 : Subsystem
  Universal Bridge : spsUniversalBridgeLib/Universal Bridge  Arms=2  SnubberResistance=0.01  SnubberCapacitance=1e-8  Device=Diodes  Ron=1e-3  Lon=0  ForwardVoltages="[  0  0  ]"  ForwardVoltage=3  GTOparameters=[ 10e-6 , 20e-6 ]  IGBTparameters=[ 1e-6 , 2e-6 ]  Measurements=None  Measurements_2=None  converterType=Rectifier
  Vm1 : spsVoltageMeasurementLib/Voltage Measurement  PhasorSimulation=off  OutputType=Complex  PSBequivalent=0
  + : PMIOPort  Side=Left
  - : PMIOPort  Port=2  Side=Left
  A : PMIOPort  Port=3  Side=Right
  B : PMIOPort  Port=4  Side=Right
  Out1 : Outport
  wires:
  Subsystem2/1(g1) -> IGBT/Diode/1
  M/1 -> Subsystem2/1(MOD)
  Vm1/1 -> Out1/1
  connections:
  Diode/LConn1 -- Universal Bridge/RConn1 -- IGBT/Diode/LConn1
  B/RConn1 -- Universal Bridge/LConn2
  A/RConn1 -- Universal Bridge/LConn1
  Diode/RConn1 -- C/LConn1 -- R/LConn1 -- Vm1/LConn1
  IGBT/Diode/RConn1 -- C/RConn1 -- R/RConn1 -- Vm1/LConn2 -- Universal Bridge/RConn2

== system DPWMA_17_Level_Rectifier_Dual_PI/Subsystem1/子模块5 ==
  M : Inport
  C : spsSeriesRLCBranchLib/Series RLC Branch  LConnTagsString=__new0  RConnTagsString=__new0  BranchType=C  Resistance=0  Inductance=0  SetiL0=off  InitialCurrent=0  Capacitance=4e-3  Setx0=on  InitialVoltage=1000  Measurements=None
  Diode : spsDiodeLib/Diode  Ron=0.001  Lon=0  Vf=2  IC=0  UseSnubber=0  Rs=1e6  Cs=2e-9  Measurements=off
  IGBT/Diode : spsIGBTDiodeLib/IGBT//Diode  Ron=1e-3  Rs=1e5  Cs=inf  Measurements=off
  R : spsSeriesRLCBranchLib/Series RLC Branch  LConnTagsString=__new0  RConnTagsString=__new0  BranchType=R  Resistance=15  Inductance=0  SetiL0=off  InitialCurrent=0  Capacitance=2e-3  Setx0=on  InitialVoltage=311  Measurements=None
  Subsystem2 : Subsystem
  Universal Bridge : spsUniversalBridgeLib/Universal Bridge  Arms=2  SnubberResistance=0.01  SnubberCapacitance=1e-8  Device=Diodes  Ron=1e-3  Lon=0  ForwardVoltages="[  0  0  ]"  ForwardVoltage=3  GTOparameters=[ 10e-6 , 20e-6 ]  IGBTparameters=[ 1e-6 , 2e-6 ]  Measurements=None  Measurements_2=None  converterType=Rectifier
  Vm1 : spsVoltageMeasurementLib/Voltage Measurement  PhasorSimulation=off  OutputType=Complex  PSBequivalent=0
  + : PMIOPort  Side=Left
  - : PMIOPort  Port=2  Side=Left
  A : PMIOPort  Port=3  Side=Right
  B : PMIOPort  Port=4  Side=Right
  Out1 : Outport
  wires:
  Vm1/1 -> Out1/1
  M/1 -> Subsystem2/1(MOD)
  Subsystem2/1(g1) -> IGBT/Diode/1
  connections:
  Universal Bridge/RConn2 -- Vm1/LConn2 -- R/RConn1 -- C/RConn1 -- IGBT/Diode/RConn1
  Vm1/LConn1 -- R/LConn1 -- C/LConn1 -- Diode/RConn1
  A/RConn1 -- Universal Bridge/LConn1
  B/RConn1 -- Universal Bridge/LConn2
  IGBT/Diode/LConn1 -- Universal Bridge/RConn1 -- Diode/LConn1

== system DPWMA_17_Level_Rectifier_Dual_PI/Subsystem1/子模块6 ==
  M : Inport
  C : spsSeriesRLCBranchLib/Series RLC Branch  LConnTagsString=__new0  RConnTagsString=__new0  BranchType=C  Resistance=0  Inductance=0  SetiL0=off  InitialCurrent=0  Capacitance=4e-3  Setx0=on  InitialVoltage=1000  Measurements=None
  Diode : spsDiodeLib/Diode  Ron=0.001  Lon=0  Vf=2  IC=0  UseSnubber=0  Rs=1e6  Cs=2e-9  Measurements=off
  IGBT/Diode : spsIGBTDiodeLib/IGBT//Diode  Ron=1e-3  Rs=1e5  Cs=inf  Measurements=off
  R : spsSeriesRLCBranchLib/Series RLC Branch  LConnTagsString=__new0  RConnTagsString=__new0  BranchType=R  Resistance=15  Inductance=0  SetiL0=off  InitialCurrent=0  Capacitance=2e-3  Setx0=on  InitialVoltage=311  Measurements=None
  Subsystem2 : Subsystem
  Universal Bridge : spsUniversalBridgeLib/Universal Bridge  Arms=2  SnubberResistance=0.01  SnubberCapacitance=1e-8  Device=Diodes  Ron=1e-3  Lon=0  ForwardVoltages="[  0  0  ]"  ForwardVoltage=3  GTOparameters=[ 10e-6 , 20e-6 ]  IGBTparameters=[ 1e-6 , 2e-6 ]  Measurements=None  Measurements_2=None  converterType=Rectifier
  Vm1 : spsVoltageMeasurementLib/Voltage Measurement  PhasorSimulation=off  OutputType=Complex  PSBequivalent=0
  + : PMIOPort  Side=Left
  - : PMIOPort  Port=2  Side=Left
  A : PMIOPort  Port=3  Side=Right
  B : PMIOPort  Port=4  Side=Right
  Out1 : Outport
  wires:
  Vm1/1 -> Out1/1
  M/1 -> Subsystem2/1(MOD)
  Subsystem2/1(g1) -> IGBT/Diode/1
  connections:
  Universal Bridge/RConn2 -- Vm1/LConn2 -- R/RConn1 -- C/RConn1 -- IGBT/Diode/RConn1
  Vm1/LConn1 -- R/LConn1 -- C/LConn1 -- Diode/RConn1
  A/RConn1 -- Universal Bridge/LConn1
  B/RConn1 -- Universal Bridge/LConn2
  IGBT/Diode/LConn1 -- Universal Bridge/RConn1 -- Diode/LConn1

== system DPWMA_17_Level_Rectifier_Dual_PI/Subsystem1/子模块7 ==
  M : Inport
  C : spsSeriesRLCBranchLib/Series RLC Branch  LConnTagsString=__new0  RConnTagsString=__new0  BranchType=C  Resistance=0  Inductance=0  SetiL0=off  InitialCurrent=0  Capacitance=4e-3  Setx0=on  InitialVoltage=1000  Measurements=None
  Diode : spsDiodeLib/Diode  Ron=0.001  Lon=0  Vf=2  IC=0  UseSnubber=0  Rs=1e6  Cs=2e-9  Measurements=off
  IGBT/Diode : spsIGBTDiodeLib/IGBT//Diode  Ron=1e-3  Rs=1e5  Cs=inf  Measurements=off
  R : spsSeriesRLCBranchLib/Series RLC Branch  LConnTagsString=__new0  RConnTagsString=__new0  BranchType=R  Resistance=15  Inductance=0  SetiL0=off  InitialCurrent=0  Capacitance=2e-3  Setx0=on  InitialVoltage=311  Measurements=None
  Subsystem2 : Subsystem
  Universal Bridge : spsUniversalBridgeLib/Universal Bridge  Arms=2  SnubberResistance=0.01  SnubberCapacitance=1e-8  Device=Diodes  Ron=1e-3  Lon=0  ForwardVoltages="[  0  0  ]"  ForwardVoltage=3  GTOparameters=[ 10e-6 , 20e-6 ]  IGBTparameters=[ 1e-6 , 2e-6 ]  Measurements=None  Measurements_2=None  converterType=Rectifier
  Vm1 : spsVoltageMeasurementLib/Voltage Measurement  PhasorSimulation=off  OutputType=Complex  PSBequivalent=0
  + : PMIOPort  Side=Left
  - : PMIOPort  Port=2  Side=Left
  A : PMIOPort  Port=3  Side=Right
  B : PMIOPort  Port=4  Side=Right
  Out1 : Outport
  wires:
  Subsystem2/1(g1) -> IGBT/Diode/1
  M/1 -> Subsystem2/1(MOD)
  Vm1/1 -> Out1/1
  connections:
  Diode/LConn1 -- Universal Bridge/RConn1 -- IGBT/Diode/LConn1
  B/RConn1 -- Universal Bridge/LConn2
  A/RConn1 -- Universal Bridge/LConn1
  Diode/RConn1 -- C/LConn1 -- R/LConn1 -- Vm1/LConn1
  IGBT/Diode/RConn1 -- C/RConn1 -- R/RConn1 -- Vm1/LConn2 -- Universal Bridge/RConn2

== system DPWMA_17_Level_Rectifier_Dual_PI/Subsystem1/子模块8 ==
  M : Inport
  C : spsSeriesRLCBranchLib/Series RLC Branch  LConnTagsString=__new0  RConnTagsString=__new0  BranchType=C  Resistance=0  Inductance=0  SetiL0=off  InitialCurrent=0  Capacitance=4e-3  Setx0=on  InitialVoltage=1000  Measurements=None
  Diode : spsDiodeLib/Diode  Ron=0.001  Lon=0  Vf=2  IC=0  UseSnubber=0  Rs=1e6  Cs=2e-9  Measurements=off
  IGBT/Diode : spsIGBTDiodeLib/IGBT//Diode  Ron=1e-3  Rs=1e5  Cs=inf  Measurements=off
  R : spsSeriesRLCBranchLib/Series RLC Branch  LConnTagsString=__new0  RConnTagsString=__new0  BranchType=R  Resistance=15  Inductance=0  SetiL0=off  InitialCurrent=0  Capacitance=2e-3  Setx0=on  InitialVoltage=311  Measurements=None
  Subsystem2 : Subsystem
  Universal Bridge : spsUniversalBridgeLib/Universal Bridge  Arms=2  SnubberResistance=0.01  SnubberCapacitance=1e-8  Device=Diodes  Ron=1e-3  Lon=0  ForwardVoltages="[  0  0  ]"  ForwardVoltage=3  GTOparameters=[ 10e-6 , 20e-6 ]  IGBTparameters=[ 1e-6 , 2e-6 ]  Measurements=None  Measurements_2=None  converterType=Rectifier
  Vm1 : spsVoltageMeasurementLib/Voltage Measurement  PhasorSimulation=off  OutputType=Complex  PSBequivalent=0
  + : PMIOPort  Side=Left
  - : PMIOPort  Port=2  Side=Left
  A : PMIOPort  Port=3  Side=Right
  B : PMIOPort  Port=4  Side=Right
  Out1 : Outport
  wires:
  Vm1/1 -> Out1/1
  M/1 -> Subsystem2/1(MOD)
  Subsystem2/1(g1) -> IGBT/Diode/1
  connections:
  Universal Bridge/RConn2 -- Vm1/LConn2 -- R/RConn1 -- C/RConn1 -- IGBT/Diode/RConn1
  Vm1/LConn1 -- R/LConn1 -- C/LConn1 -- Diode/RConn1
  A/RConn1 -- Universal Bridge/LConn1
  B/RConn1 -- Universal Bridge/LConn2
  IGBT/Diode/LConn1 -- Universal Bridge/RConn1 -- Diode/LConn1

== system DPWMA_17_Level_Rectifier_Dual_PI/Subsystem2/子模块1 ==
  M : Inport
  C : spsSeriesRLCBranchLib/Series RLC Branch  LConnTagsString=__new0  RConnTagsString=__new0  BranchType=C  Resistance=0  Inductance=0  SetiL0=off  InitialCurrent=0  Capacitance=4e-3  Setx0=on  InitialVoltage=1000  Measurements=None
  Diode : spsDiodeLib/Diode  Ron=0.001  Lon=0  Vf=2  IC=0  UseSnubber=0  Rs=1e6  Cs=2e-9  Measurements=off
  IGBT/Diode : spsIGBTDiodeLib/IGBT//Diode  Ron=1e-3  Rs=1e5  Cs=inf  Measurements=off
  R : spsSeriesRLCBranchLib/Series RLC Branch  LConnTagsString=__new0  RConnTagsString=__new0  BranchType=R  Resistance=15  Inductance=0  SetiL0=off  InitialCurrent=0  Capacitance=2e-3  Setx0=on  InitialVoltage=311  Measurements=None
  Subsystem2 : Subsystem
  Universal Bridge : spsUniversalBridgeLib/Universal Bridge  Arms=2  SnubberResistance=0.01  SnubberCapacitance=1e-8  Device=Diodes  Ron=1e-3  Lon=0  ForwardVoltages="[  0  0  ]"  ForwardVoltage=3  GTOparameters=[ 10e-6 , 20e-6 ]  IGBTparameters=[ 1e-6 , 2e-6 ]  Measurements=None  Measurements_2=None  converterType=Rectifier
  Vm1 : spsVoltageMeasurementLib/Voltage Measurement  PhasorSimulation=off  OutputType=Complex  PSBequivalent=0
  + : PMIOPort  Side=Left
  - : PMIOPort  Port=2  Side=Left
  A : PMIOPort  Port=3  Side=Right
  B : PMIOPort  Port=4  Side=Right
  Out1 : Outport
  wires:
  Vm1/1 -> Out1/1
  M/1 -> Subsystem2/1(MOD)
  Subsystem2/1(g1) -> IGBT/Diode/1
  connections:
  Universal Bridge/RConn2 -- Vm1/LConn2 -- R/RConn1 -- C/RConn1 -- IGBT/Diode/RConn1
  Vm1/LConn1 -- R/LConn1 -- C/LConn1 -- Diode/RConn1
  A/RConn1 -- Universal Bridge/LConn1
  B/RConn1 -- Universal Bridge/LConn2
  IGBT/Diode/LConn1 -- Universal Bridge/RConn1 -- Diode/LConn1

== system DPWMA_17_Level_Rectifier_Dual_PI/Subsystem2/子模块2 ==
  M : Inport
  C : spsSeriesRLCBranchLib/Series RLC Branch  LConnTagsString=__new0  RConnTagsString=__new0  BranchType=C  Resistance=0  Inductance=0  SetiL0=off  InitialCurrent=0  Capacitance=4e-3  Setx0=on  InitialVoltage=1000  Measurements=None
  Diode : spsDiodeLib/Diode  Ron=0.001  Lon=0  Vf=2  IC=0  UseSnubber=0  Rs=1e6  Cs=2e-9  Measurements=off
  IGBT/Diode : spsIGBTDiodeLib/IGBT//Diode  Ron=1e-3  Rs=1e5  Cs=inf  Measurements=off
  R : spsSeriesRLCBranchLib/Series RLC Branch  LConnTagsString=__new0  RConnTagsString=__new0  BranchType=R  Resistance=15  Inductance=0  SetiL0=off  InitialCurrent=0  Capacitance=2e-3  Setx0=on  InitialVoltage=311  Measurements=None
  Subsystem2 : Subsystem
  Universal Bridge : spsUniversalBridgeLib/Universal Bridge  Arms=2  SnubberResistance=0.01  SnubberCapacitance=1e-8  Device=Diodes  Ron=1e-3  Lon=0  ForwardVoltages="[  0  0  ]"  ForwardVoltage=3  GTOparameters=[ 10e-6 , 20e-6 ]  IGBTparameters=[ 1e-6 , 2e-6 ]  Measurements=None  Measurements_2=None  converterType=Rectifier
  Vm1 : spsVoltageMeasurementLib/Voltage Measurement  PhasorSimulation=off  OutputType=Complex  PSBequivalent=0
  + : PMIOPort  Side=Left
  - : PMIOPort  Port=2  Side=Left
  A : PMIOPort  Port=3  Side=Right
  B : PMIOPort  Port=4  Side=Right
  Out1 : Outport
  wires:
  Vm1/1 -> Out1/1
  M/1 -> Subsystem2/1(MOD)
  Subsystem2/1(g1) -> IGBT/Diode/1
  connections:
  Universal Bridge/RConn2 -- Vm1/LConn2 -- R/RConn1 -- C/RConn1 -- IGBT/Diode/RConn1
  Vm1/LConn1 -- R/LConn1 -- C/LConn1 -- Diode/RConn1
  A/RConn1 -- Universal Bridge/LConn1
  B/RConn1 -- Universal Bridge/LConn2
  IGBT/Diode/LConn1 -- Universal Bridge/RConn1 -- Diode/LConn1

== system DPWMA_17_Level_Rectifier_Dual_PI/Subsystem2/子模块3 ==
  M : Inport
  C : spsSeriesRLCBranchLib/Series RLC Branch  LConnTagsString=__new0  RConnTagsString=__new0  BranchType=C  Resistance=0  Inductance=0  SetiL0=off  InitialCurrent=0  Capacitance=4e-3  Setx0=on  InitialVoltage=1000  Measurements=None
  Diode : spsDiodeLib/Diode  Ron=0.001  Lon=0  Vf=2  IC=0  UseSnubber=0  Rs=1e6  Cs=2e-9  Measurements=off
  IGBT/Diode : spsIGBTDiodeLib/IGBT//Diode  Ron=1e-3  Rs=1e5  Cs=inf  Measurements=off
  R : spsSeriesRLCBranchLib/Series RLC Branch  LConnTagsString=__new0  RConnTagsString=__new0  BranchType=R  Resistance=15  Inductance=0  SetiL0=off  InitialCurrent=0  Capacitance=2e-3  Setx0=on  InitialVoltage=311  Measurements=None
  Subsystem2 : Subsystem
  Universal Bridge : spsUniversalBridgeLib/Universal Bridge  Arms=2  SnubberResistance=0.01  SnubberCapacitance=1e-8  Device=Diodes  Ron=1e-3  Lon=0  ForwardVoltages="[  0  0  ]"  ForwardVoltage=3  GTOparameters=[ 10e-6 , 20e-6 ]  IGBTparameters=[ 1e-6 , 2e-6 ]  Measurements=None  Measurements_2=None  converterType=Rectifier
  Vm1 : spsVoltageMeasurementLib/Voltage Measurement  PhasorSimulation=off  OutputType=Complex  PSBequivalent=0
  + : PMIOPort  Side=Left
  - : PMIOPort  Port=2  Side=Left
  A : PMIOPort  Port=3  Side=Right
  B : PMIOPort  Port=4  Side=Right
  Out1 : Outport
  wires:
  Subsystem2/1(g1) -> IGBT/Diode/1
  M/1 -> Subsystem2/1(MOD)
  Vm1/1 -> Out1/1
  connections:
  Diode/LConn1 -- Universal Bridge/RConn1 -- IGBT/Diode/LConn1
  B/RConn1 -- Universal Bridge/LConn2
  A/RConn1 -- Universal Bridge/LConn1
  Diode/RConn1 -- C/LConn1 -- R/LConn1 -- Vm1/LConn1
  IGBT/Diode/RConn1 -- C/RConn1 -- R/RConn1 -- Vm1/LConn2 -- Universal Bridge/RConn2

== system DPWMA_17_Level_Rectifier_Dual_PI/Subsystem2/子模块4 ==
  M : Inport
  C : spsSeriesRLCBranchLib/Series RLC Branch  LConnTagsString=__new0  RConnTagsString=__new0  BranchType=C  Resistance=0  Inductance=0  SetiL0=off  InitialCurrent=0  Capacitance=4e-3  Setx0=on  InitialVoltage=1000  Measurements=None
  Diode : spsDiodeLib/Diode  Ron=0.001  Lon=0  Vf=2  IC=0  UseSnubber=0  Rs=1e6  Cs=2e-9  Measurements=off
  IGBT/Diode : spsIGBTDiodeLib/IGBT//Diode  Ron=1e-3  Rs=1e5  Cs=inf  Measurements=off
  R : spsSeriesRLCBranchLib/Series RLC Branch  LConnTagsString=__new0  RConnTagsString=__new0  BranchType=R  Resistance=15  Inductance=0  SetiL0=off  InitialCurrent=0  Capacitance=2e-3  Setx0=on  InitialVoltage=311  Measurements=None
  Subsystem2 : Subsystem
  Universal Bridge : spsUniversalBridgeLib/Universal Bridge  Arms=2  SnubberResistance=0.01  SnubberCapacitance=1e-8  Device=Diodes  Ron=1e-3  Lon=0  ForwardVoltages="[  0  0  ]"  ForwardVoltage=3  GTOparameters=[ 10e-6 , 20e-6 ]  IGBTparameters=[ 1e-6 , 2e-6 ]  Measurements=None  Measurements_2=None  converterType=Rectifier
  Vm1 : spsVoltageMeasurementLib/Voltage Measurement  PhasorSimulation=off  OutputType=Complex  PSBequivalent=0
  + : PMIOPort  Side=Left
  - : PMIOPort  Port=2  Side=Left
  A : PMIOPort  Port=3  Side=Right
  B : PMIOPort  Port=4  Side=Right
  Out1 : Outport
  wires:
  Vm1/1 -> Out1/1
  M/1 -> Subsystem2/1(MOD)
  Subsystem2/1(g1) -> IGBT/Diode/1
  connections:
  Universal Bridge/RConn2 -- Vm1/LConn2 -- R/RConn1 -- C/RConn1 -- IGBT/Diode/RConn1
  Vm1/LConn1 -- R/LConn1 -- C/LConn1 -- Diode/RConn1
  A/RConn1 -- Universal Bridge/LConn1
  B/RConn1 -- Universal Bridge/LConn2
  IGBT/Diode/LConn1 -- Universal Bridge/RConn1 -- Diode/LConn1

== system DPWMA_17_Level_Rectifier_Dual_PI/Subsystem2/子模块5 ==
  M : Inport
  C : spsSeriesRLCBranchLib/Series RLC Branch  LConnTagsString=__new0  RConnTagsString=__new0  BranchType=C  Resistance=0  Inductance=0  SetiL0=off  InitialCurrent=0  Capacitance=4e-3  Setx0=on  InitialVoltage=1000  Measurements=None
  Diode : spsDiodeLib/Diode  Ron=0.001  Lon=0  Vf=2  IC=0  UseSnubber=0  Rs=1e6  Cs=2e-9  Measurements=off
  IGBT/Diode : spsIGBTDiodeLib/IGBT//Diode  Ron=1e-3  Rs=1e5  Cs=inf  Measurements=off
  R : spsSeriesRLCBranchLib/Series RLC Branch  LConnTagsString=__new0  RConnTagsString=__new0  BranchType=R  Resistance=15  Inductance=0  SetiL0=off  InitialCurrent=0  Capacitance=2e-3  Setx0=on  InitialVoltage=311  Measurements=None
  Subsystem2 : Subsystem
  Universal Bridge : spsUniversalBridgeLib/Universal Bridge  Arms=2  SnubberResistance=0.01  SnubberCapacitance=1e-8  Device=Diodes  Ron=1e-3  Lon=0  ForwardVoltages="[  0  0  ]"  ForwardVoltage=3  GTOparameters=[ 10e-6 , 20e-6 ]  IGBTparameters=[ 1e-6 , 2e-6 ]  Measurements=None  Measurements_2=None  converterType=Rectifier
  Vm1 : spsVoltageMeasurementLib/Voltage Measurement  PhasorSimulation=off  OutputType=Complex  PSBequivalent=0
  + : PMIOPort  Side=Left
  - : PMIOPort  Port=2  Side=Left
  A : PMIOPort  Port=3  Side=Right
  B : PMIOPort  Port=4  Side=Right
  Out1 : Outport
  wires:
  Subsystem2/1(g1) -> IGBT/Diode/1
  M/1 -> Subsystem2/1(MOD)
  Vm1/1 -> Out1/1
  connections:
  Diode/LConn1 -- Universal Bridge/RConn1 -- IGBT/Diode/LConn1
  B/RConn1 -- Universal Bridge/LConn2
  A/RConn1 -- Universal Bridge/LConn1
  Diode/RConn1 -- C/LConn1 -- R/LConn1 -- Vm1/LConn1
  IGBT/Diode/RConn1 -- C/RConn1 -- R/RConn1 -- Vm1/LConn2 -- Universal Bridge/RConn2
